simulink model "aula_10"  (R2024a)
settings: Solver=VariableStepAuto  StartTime=0.0  StopTime=tsim  MaxStep=1e-1  RelTol=1e-3
values from neighbouring files (symbols this model uses):
  ae0 = 0.6    [Lab11.m]    (also in Lab11_pronto.m; Lab_7.m; aula08.m; aula08_lab.m)
  as0 = 0.5    [Lab11.m]    (also in Lab11_pronto.m; Lab_7.m; aula08.m; aula08_lab.m)
  b = 0.5    [Lab11.m]    (also in Lab11_pronto.m)
  c = 0    [Lab11.m]    (also in Lab11_pronto.m)
  gamma = 1/8    (= 0.125)    [Lab11.m]    (also in Lab11_pronto.m; aula08.m; aula08_lab.m; lab09.m)
  H0 = ((ke*ae0)/(ks*as0*sqrt(2*g)))^2    [Lab11.m]    (also in Lab11_pronto.m = ((ke*ae0)/(ks*as0*sqrt(2*gg)))^2; Lab_7.m; aula08.m; aula08_lab.m)
  H_ref = H0 + 0.10    [Lab11_pronto.m]    (also in Lab_7.m; aula08.m; aula08_lab.m)
  Kc = 0.2587    [Lab11.m]    (also in Lab11_pronto.m; aula08.m = 3; aula08_lab.m = 1; lab09.m = M(idx).Kc)
  Td = 20.66    [Lab11.m]    (also in Lab11_pronto.m; aula08.m = 0; aula08_lab.m = 0; lab09.m = M(idx).Td)
  theta = 2*tau    (= 54.42)    [Lab11.m]    (also in Lab11_pronto.m; lab09.m = 136.05)
  Ti = 53.90    (= 53.9)    [Lab11.m]    (also in Lab11_pronto.m; aula08.m = 1.2; aula08_lab.m = 20; lab09.m = M(idx).Ti)
  tsim = 2500    [Lab11.m]    (also in Lab11_pronto.m; Lab_7.m = 500; aula08.m = 500; aula08_lab.m = 500)
libraries: cstblocks x2, slpidlib x1
settings Model: Creator=Prof. Daniel Cruz  LastModifiedBy=Prof. Daniel Cruz
settings SolverCC: AlgebraicLoopSolver=TrustRegion
settings DebuggingCC: UnconnectedInputMsg=warning  UnconnectedOutputMsg=warning  UnconnectedLineMsg=warning
settings ModelReferenceCC: EnableRefExpFcnMdlSchedulingChecks=on
settings RTWCC: GPUComputeCapability=3.5

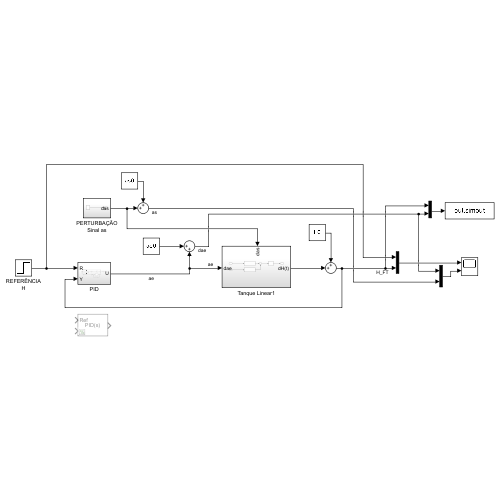
[thumbnail: Simulink's stored preview of the top-level diagram]
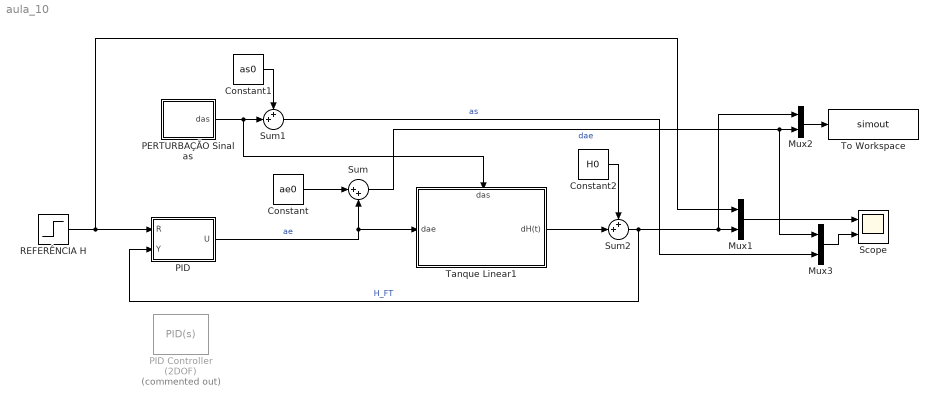
== system aula_10 ==
  Constant : Constant  Value=ae0
  Constant1 : Constant  Value=as0
  Constant2 : Constant  Value=H0
  Mux1 : Mux  Inputs=2
  Mux2 : Mux  Inputs=2
  Mux3 : Mux  Inputs=2
  PERTURBAÇÃO Sinal as : Subsystem
  PID : Subsystem
  PID Controller (2DOF) : slpidlib/PID Controller (2DOF)  Commented=on  Controller=PID  Form=Ideal  TimeDomain=Continuous-time  UseExternalTs=off  SampleTime=-1  IntegratorMethod=Forward Euler  FilterMethod=Forward Euler  ControllerParametersSource=internal  P=Kc  I=1/Ti  UseKiTs=off  D=Td  UseExternalDerivativeSource=off  N=1/(gamma*Td)  UseFilter=on  b=1  c=1  TunerSelectOption=Transfer Function Based (PID Tuner App)  InitialConditionSource=internal  InitialConditionForIntegrator=0  InitialConditionForFilter=0  DifferentiatorICPrevScaledInput=0  ExternalReset=none  TrackingMode=off  Kt=1  LimitOutput=off  SatLimitsSource=internal  UpperSaturationLimit=inf  LowerSaturationLimit=-inf  LinearizeAsGain=on  AntiWindupMode=none  Kb=1  LimitIntegrator=off  UpperIntegratorSaturationLimit=inf  LowerIntegratorSaturationLimit=-inf  POutMin=[]  POutMax=[]  IOutMin=[]  IOutMax=[]  DOutMin=[]  DOutMax=[]  NOutMin=[]  NOutMax=[]  bOutMin=[]  bOutMax=[]  cOutMin=[]  cOutMax=[]  SumOutMin=[]  SumOutMax=[]  SaturationOutMin=[]  SaturationOutMax=[]  PParamMin=[]  PParamMax=[]  IParamMin=[]  IParamMax=[]  DParamMin=[]  DParamMax=[]  NParamMin=[]  NParamMax=[]  bParamMin=[]  bParamMax=[]  cParamMin=[]  cParamMax=[]  KbParamMin=[]  KbParamMax=[]  KtParamMin=[]  KtParamMax=[]  KbOutMin=[]  KbOutMax=[]  KtOutMin=[]  KtOutMax=[]  IntegratorOutMin=[]  IntegratorOutMax=[]  FilterOutMin=[]  FilterOutMax=[]  SumI1OutMin=[]  SumI1OutMax=[]  SumI2OutMin=[]  SumI2OutMax=[]  SumI3OutMin=[]  SumI3OutMax=[]  SumI4OutMin=[]  SumI4OutMax=[]  SumDOutMin=[]  SumDOutMax=[]  Sum1OutMin=[]  Sum1OutMax=[]  Sum2OutMin=[]  Sum2OutMax=[]  Sum3OutMin=[]  Sum3OutMax=[]  DifferentiatorOutMin=[]  DifferentiatorOutMax=[]  FilterDiffOutCoefMin=[]  FilterDiffOutCoefMax=[]  ReciprocalOutMin=[]  ReciprocalOutMax=[]  SumDenOutMin=[]  SumDenOutMax=[]  SumNumOutMin=[]  SumNumOutMax=[]  DivideOutMin=[]  DivideOutMax=[]  UdiffTsProdOutMin=[]  UdiffTsProdOutMax=[]  NTsProdOutMin=[]  NTsProdOutMax=[]  UintegralTsProdOutMin=[]  UintegralTsProdOutMax=[]  UngainTsProdOutMin=[]  UngainTsProdOutMax=[]  ClampingZeroOutDataTypeStr=Inherit: Inherit via back propagation  ClampingZeroOutMin=[]  ClampingZeroOutMax=[]  FilterDenConstantOutDataTypeStr=Inherit: Inherit via back propagation  FilterDenConstantOutMin=[]  FilterDenConstantOutMax=[]  PCopyOutDataTypeStr=Inherit: Inherit via back propagation  PCopyOutMin=[]  PCopyOutMax=[]  NCopyOutDataTypeStr=Inherit: Inherit via back propagation  NCopyOutMin=[]  NCopyOutMax=[]  IntegratorContinuousStateAttributes=''  IntegratorStateMustResolveToSignalObject=off  IntegratorRTWStateStorageClass=Auto  FilterContinuousStateAttributes=''  FilterStateMustResolveToSignalObject=off  FilterRTWStateStorageClass=Auto  ParallelPVariant=Passthrough  IdealPVariant=InternalParameters  IVariant=InternalParameters  DVariant=InternalParameters  bVariant=InternalParameters  cVariant=InternalParameters  IntegratorVariant=Continuous  SatVariant=Disabled  AWVariant=Passthrough  PCopyVariant=Disabled  TRVariant=Disabled  FdbkBlocksVariant=Forward  IdealPFdbkVariant=Disabled  SatFdbkVariant=Disabled  DerivativeFilterVariant=ContFilter  NVariant=InternalParameters  NCopyVariant=Disabled  FilterICVariant=InternalICsFilter  IntegratorICVariant=InternalICs  ExternalResetVariant=Disabled  TRSumVariant=Passthrough  SumFdbkVariant=Disabled  SumVariant=Sum_PID  TsampFilterVariant=InternalTs  TsampNgainVariant=Passthrough  TsampIntegralVariant=Disabled_SignalSpec  ExternalSaturationOutDataTypeStr=Inherit: Same as second input  DerivativeSourceVariant=ErrorSignal
  REFERÊNCIA H : Step  Time=0  Before=H0  After=H_ref  SampleTime=0
  Scope : Scope  NumInputPorts=2
  Sum : Sum  Inputs=|++
  Sum1 : Sum  Inputs=++|
  Sum2 : Sum  Inputs=++|
  Tanque Linear1 : Subsystem
      settings: PortSchema="{\"entries\":[{\"content\":{\"sides\":[{\"content\":{\"connectorIds\":[\"In1\"]},\"type\":\"ConnectorPlacement.EquallySpacedRectSide\",\"uuid\":\"f67b16a6-d13c-4ce1-92bf-a3b7b78f55b2\"},{\"content\":{\"connectorIds\":[\"Out1\"],\"side\":\"RIGHT\"},\"type\":\"ConnectorPlacement.EquallySpacedRectSide\",\"uuid\":\"6dfa0371-c497-4466-b77b-e5c5fe181385\"},{\"content\":{\"connectorIds\":[\"In2\"],\"side\":\"TOP\"},\"type\":\"ConnectorPlacement.EquallySpacedRectSide\",\"uuid\":\"6450f77e-1436-4798-86e5-b0a6495bdb9b\"}]},\"type\":\"ConnectorPlacement.EquallySpacedConnector\",\"uuid\":\"6402b57b-709e-4d3a-bcb1-330d3ba010a6\"}],\"packageUris\":[\"http://schema.mathworks.com/mf0/Connector/R2020b\"],\"version\":\"1.0\"}"
  To Workspace : ToWorkspace  VariableName=simout  SaveFormat=Timeseries  SampleTime=-1
  wires:
  Constant/1 -> Sum/1
  Constant1/1 -> Sum1/1
  PERTURBAÇÃO Sinal as/1(das) -> Tanque Linear1/2(das), Sum1/2
  Tanque Linear1/1(dH(t)) -> Sum2/2
  Constant2/1 -> Sum2/1
  Sum2/1 -> PID/2(Y), Mux2/1, Mux1/2  "H_FT"
  Mux1/1 -> Scope/1
  Sum1/1 -> Mux3/2  "as"
  REFERÊNCIA H/1 -> PID/1(R), Mux1/1
  PID/1(U) -> Tanque Linear1/1(dae), Sum/2  "ae"
  Mux2/1 -> To Workspace/1
  Mux3/1 -> Scope/2
  Sum/1 -> Mux3/1, Mux2/2  "dae"

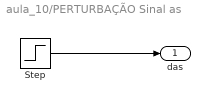
== system aula_10/PERTURBAÇÃO Sinal as ==
  Step : Step  Time=(4/8)*tsim  After=0.1  SampleTime=0
  das : Outport
  wires:
  Step/1 -> das/1

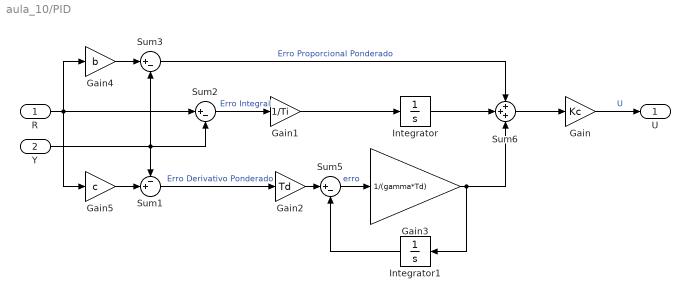
== system aula_10/PID ==
  R : Inport
  Y : Inport  Port=2
  Gain : Gain  Gain=Kc
  Gain1 : Gain  Gain=1/Ti
  Gain2 : Gain  Gain=Td
  Gain3 : Gain  Gain=1/(gamma*Td)
  Gain4 : Gain  Gain=b
  Gain5 : Gain  Gain=c
  Integrator : Integrator
  Integrator1 : Integrator
  Sum1 : Sum  Inputs=-+|
  Sum2 : Sum  Inputs=|+-
  Sum3 : Sum  Inputs=|+-
  Sum5 : Sum  Inputs=|+-
  Sum6 : Sum  Inputs=+++
  U : Outport
  wires:
  Gain2/1 -> Sum5/1
  Gain3/1 -> Sum6/3, Integrator1/1
  Integrator1/1 -> Sum5/2
  Integrator/1 -> Sum6/2
  Sum5/1 -> Gain3/1  "erro"
  Sum6/1 -> Gain/1
  Gain1/1 -> Integrator/1
  R/1 -> Sum2/1, Gain4/1, Gain5/1
  Y/1 -> Sum1/1, Sum2/2, Sum3/2
  Gain/1 -> U/1  "U"
  Gain4/1 -> Sum3/1
  Sum3/1 -> Sum6/1  "Erro Proporcional Ponderado"
  Gain5/1 -> Sum1/2
  Sum2/1 -> Gain1/1  "Erro Integral"
  Sum1/1 -> Gain2/1  "Erro Derivativo Ponderado"

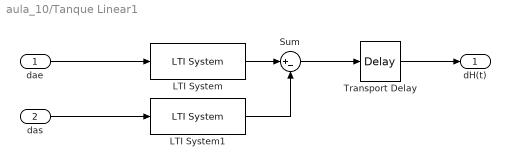
== system aula_10/Tanque Linear1 ==
  dae : Inport
  das : Inport  Port=2
  LTI System : cstblocks/LTI System  sys=G  IC=[]  PadeOrder=0
  LTI System1 : cstblocks/LTI System  sys=Gas  IC=[]  PadeOrder=0
  Sum : Sum  Inputs=|+-
  Transport Delay : TransportDelay  DelayTime=theta
  dH(t) : Outport
  wires:
  dae/1 -> LTI System/1
  das/1 -> LTI System1/1
  LTI System/1 -> Sum/1
  LTI System1/1 -> Sum/2
  Sum/1 -> Transport Delay/1
  Transport Delay/1 -> dH(t)/1
